simulink model "g1_walking"  (R2025b)
settings: Solver=daessc  StartTime=0.0  StopTime=4.8  MaxStep=0.0005  RelTol=1e-6  AbsTol=1e-8
model workspace (MAT data in the model file):
  g1_base_p0 = [0; 0; 0.8]
  g1_base_rpy0 = [0; 0; 0]
  g1_command_height = 0.8
  g1_forward_command = 0.1
  g1_gravity = [0 0 -9.81]
  g1_q0 = [-0.05; 0; 0; -0.05; 0; 0; 0.1; 0; 0; 0; 0; 0; 0; -0.05; 0; 0; -0.05; 0; 0; 0.1; 0; 0; 0; 0; 0; 0; 0; 0; 0]
  g1_qd0 = [0; 0; 0; 0; 0; 0; 0; 0; 0; 0; 0; 0; 0; 0; 0; 0; 0; 0; 0; 0; 0; 0; 0; 0; 0; 0; 0; 0; 0]
  g1_standing = 0
values from neighbouring files (symbols this model uses):
  g1_action_Ts = 0.002    [g1_data.sldd]
  g1_contact_threshold = 1.0    [g1_data.sldd]
  g1_cop_threshold = 5.0    [g1_data.sldd]
  g1_drive_Ts = 0.0005    [g1_data.sldd]
  g1_ground_height = 0.0    [g1_data.sldd]
  g1_limits = -0.87267 -0.2618 -1.0472 -2.5307 -0.5236 -2.7576 -0.087267 -3.0892 -1.5882 -2.618 -1.614429558 -1.972222054 -1.614429558 -0.87267 -0.2618 -1.0472 -2.5307 -2.9671 -2.7576 -0.087267 -3.0892 -2.2515 -2.618 -1.614429558 -1.972222054 -1.614429558 -0.52 -0.52 -2.618 0.5236 0.2618 2.0944 2.8798 2.9671 2.7576 2.8798 2.6704 2.2515 2.618 1.614429558 1.972222054 1.614429558 0.5236 0.2618 2.0944 2.8798 0.5236    [g1_data.sldd]
  g1_tau_max = 50.0 50.0 25.0 88.0 88.0 88.0 139.0 25.0 25.0 25.0 5.0 25.0 5.0 50.0 50.0 25.0 88.0 88.0 88.0 139.0 25.0 25.0 25.0 5.0 25.0 5.0 50.0 50.0 88.0    [g1_data.sldd]
undefined symbols (not defined in the file or in its folder): X, Y, Z
libraries: sm_lib x336, nesl_utility x122, simulink x1
(part 1 of 7)
Description:
  | Shared plant and drive model. Replace Planner and ReferenceGait model references through g1.walkingSimulation. Planner output 4 is RobotJointAction; output 3 is formulation-specific diagnostics.
settings Model: DataDictionary=g1_data.sldd  EnableAccessToBaseWorkspace=off  Creator=enoch  LastModifiedBy=enoch
settings DataIOCC: OutputOption=SpecifiedOutputTimes  OutputTimes=0:g1_drive_Ts:0.02

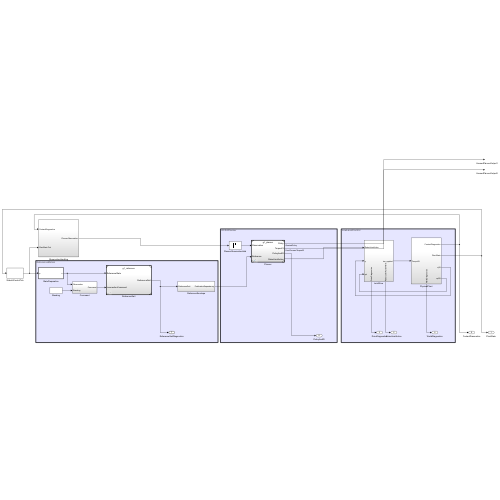
[thumbnail: Simulink's stored preview of the top-level diagram]
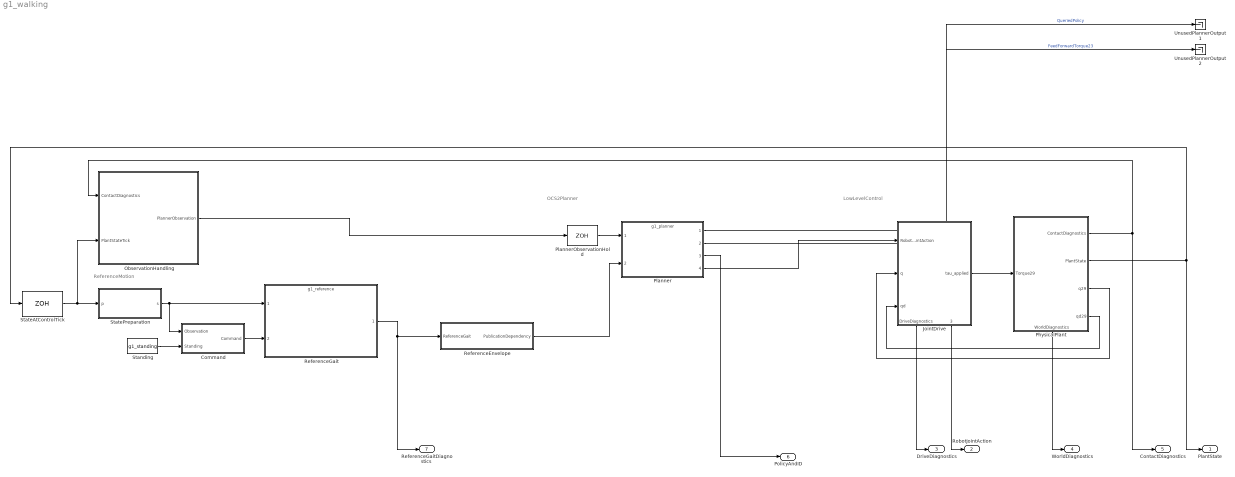
== system g1_walking ==
  note: ReferenceMotion
  note: LowLevelControl
  note: OCS2Planner
  Command : Subsystem
  JointDrive : Subsystem
      settings: PortSchema="{\"entries\":[{\"content\":{\"sides\":[{\"content\":{\"connectorIds\":[\"In1\",\"In2\",\"In3\"]},\"type\":\"ConnectorPlacement.EquallySpacedRectSide\",\"uuid\":\"f196539c-7e0c-46e2-93d7-b8c004bee5d8\"},{\"content\":{\"connectorIds\":[\"Out1\"],\"side\":\"RIGHT\"},\"type\":\"ConnectorPlacement.EquallySpacedRectSide\",\"uuid\":\"4b73e834-ba5b-4df9-9b66-b747ae678424\"},{\"content\":{\"side\":\"TOP\"},\"type\":\"ConnectorPlacement.EquallySpacedRectSide\",\"uuid\":\"8c147668-cc90-4ba0-ab32-ff0289ec25b5\"},{\"content\":{\"connectorIds\":[\"Out2\",\"Out3\"],\"side\":\"BOTTOM\"},\"type\":\"ConnectorPlacement.EquallySpacedRectSide\",\"uuid\":\"b0799187-69af-40f2-9cd9-a207ec5d2f97\"}]},\"type\":\"ConnectorPlacement.EquallySpacedConnector\",\"uuid\":\"1593d681-e81c-4265-8f53-8017c9fb3c0e\"}],\"packageUris\":[\"http://schema.mathworks.com/mf0/Connector/R2020b\"],\"version\":\"1.0\"}"
  ObservationHandling : Subsystem
  PhysicalPlant : Subsystem
      settings: PortSchema="{\"entries\":[{\"content\":{\"sides\":[{\"content\":{\"connectorIds\":[\"In1\"]},\"type\":\"ConnectorPlacement.EquallySpacedRectSide\",\"uuid\":\"a507f4f5-ee15-4ea4-b4de-ee914fc00dbd\"},{\"content\":{\"connectorIds\":[\"Out1\",\"Out2\",\"Out3\",\"Out4\"],\"side\":\"RIGHT\"},\"type\":\"ConnectorPlacement.EquallySpacedRectSide\",\"uuid\":\"97922e05-916d-4b63-ade6-e6a31880c11e\"},{\"content\":{\"side\":\"TOP\"},\"type\":\"ConnectorPlacement.EquallySpacedRectSide\",\"uuid\":\"4b0f9a05-b660-4a8d-9924-e10bf0b50292\"},{\"content\":{\"connectorIds\":[\"Out5\"],\"side\":\"BOTTOM\"},\"type\":\"ConnectorPlacement.EquallySpacedRectSide\",\"uuid\":\"154f9ed9-5c0e-4660-9782-88fd8999bb78\"}]},\"type\":\"ConnectorPlacement.EquallySpacedConnector\",\"uuid\":\"39aad6ea-4337-4531-a906-2cb26f9d93f7\"}],\"packageUris\":[\"http://schema.mathworks.com/mf0/Connector/R2020b\"],\"version\":\"1.0\"}"
  Planner : ModelReference  ModelNameDialog=g1_planner  SimulationMode=Normal  ModelReferenceVersion=1.16
  PlannerObservationHold : ZeroOrderHold  SampleTime=.002
  ReferenceEnvelope : Subsystem  Description=Flatten the coherent reference bus for the direct in-process planner call. No transport or file publication.
  ReferenceGait : ModelReference  Description=Authoritative command processing, target generation and gait state machine.  ModelNameDialog=g1_reference  SimulationMode=Normal  ModelReferenceVersion=1.19
  Standing : Constant  Value=g1_standing
  StateAtControlTick : ZeroOrderHold  SampleTime=.002
  StatePreparation : MATLAB Function  TreatAsAtomicUnit=on
  UnusedPlannerOutput1 : Terminator
  UnusedPlannerOutput2 : Terminator
  PlantState : Outport
  RobotJointAction : Outport  Port=2
  DriveDiagnostics : Outport  Port=3
  WorldDiagnostics : Outport  Port=4
  ContactDiagnostics : Outport  Port=5
  PolicyAndID : Outport  Port=6
  ReferenceGaitDiagnostics : Outport  Port=7  OutDataTypeStr=Bus: ReferenceGait  BusOutputAsStruct=on
  wires:
  PhysicalPlant/2(PlantState) -> StateAtControlTick/1, PlantState/1
  StateAtControlTick/1 -> ObservationHandling/2(PlantStateTick), StatePreparation/1(p)
  StatePreparation/1(s) -> ReferenceGait/1, Command/1(Observation)
  Standing/1 -> Command/2(Standing)
  Command/1(Command) -> ReferenceGait/2
  PhysicalPlant/1(ContactDiagnostics) -> ContactDiagnostics/1, ObservationHandling/1(ContactDiagnostics)
  PhysicalPlant/3(q29) -> JointDrive/2(q)
  PhysicalPlant/4(qd29) -> JointDrive/3(qd)
  JointDrive/1(tau_applied) -> PhysicalPlant/1(Torque29)
  JointDrive/3(RobotJointActionHeld) -> RobotJointAction/1
  JointDrive/2(DriveDiagnostics) -> DriveDiagnostics/1
  PhysicalPlant/5(WorldDiagnostics) -> WorldDiagnostics/1
  Planner/3 -> PolicyAndID/1
  ReferenceEnvelope/1(PublicationDependency) -> Planner/2
  PlannerObservationHold/1 -> Planner/1
  ObservationHandling/1(PlannerObservation) -> PlannerObservationHold/1
  ReferenceGait/1 -> ReferenceEnvelope/1(ReferenceGait), ReferenceGaitDiagnostics/1
  Planner/4 -> JointDrive/1(RobotJointAction)
  Planner/1 -> UnusedPlannerOutput1/1  "QueriedPolicy"
  Planner/2 -> UnusedPlannerOutput2/1  "FeedForwardTorque23"

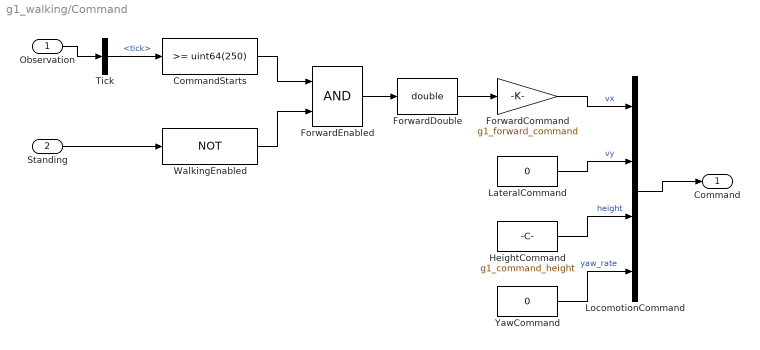
== system g1_walking/Command ==
  Observation : Inport  OutDataTypeStr=Bus: ReferenceObservation
  Standing : Inport  Port=2
  CommandStarts : simulink/Logic and Bit Operations/Compare To Constant  relop=>=  const=uint64(250)  OutDataTypeStr=boolean
  ForwardCommand : Gain  Gain=g1_forward_command
  ForwardDouble : DataTypeConversion  OutDataTypeStr=double  SaturateOnIntegerOverflow=off  RndMeth=Floor
  ForwardEnabled : Logic  AllPortsSameDT=off  OutDataTypeStr=boolean
  HeightCommand : Constant  Value=g1_command_height
  LateralCommand : Constant  Value=0
  LocomotionCommand : BusCreator  Inputs=4  OutDataTypeStr=Bus: LocomotionCommand  NonVirtualBus=on
  Tick : BusSelector  OutputSignals=tick
  WalkingEnabled : Logic  Operator=NOT  Inputs=1  AllPortsSameDT=off  OutDataTypeStr=boolean
  YawCommand : Constant  Value=0
  Command : Outport
  wires:
  Observation/1 -> Tick/1
  Tick/1 -> CommandStarts/1  "<tick>"
  Standing/1 -> WalkingEnabled/1
  CommandStarts/1 -> ForwardEnabled/1
  WalkingEnabled/1 -> ForwardEnabled/2
  ForwardEnabled/1 -> ForwardDouble/1
  ForwardDouble/1 -> ForwardCommand/1
  LocomotionCommand/1 -> Command/1
  ForwardCommand/1 -> LocomotionCommand/1  "vx"
  LateralCommand/1 -> LocomotionCommand/2  "vy"
  HeightCommand/1 -> LocomotionCommand/3  "height"
  YawCommand/1 -> LocomotionCommand/4  "yaw_rate"

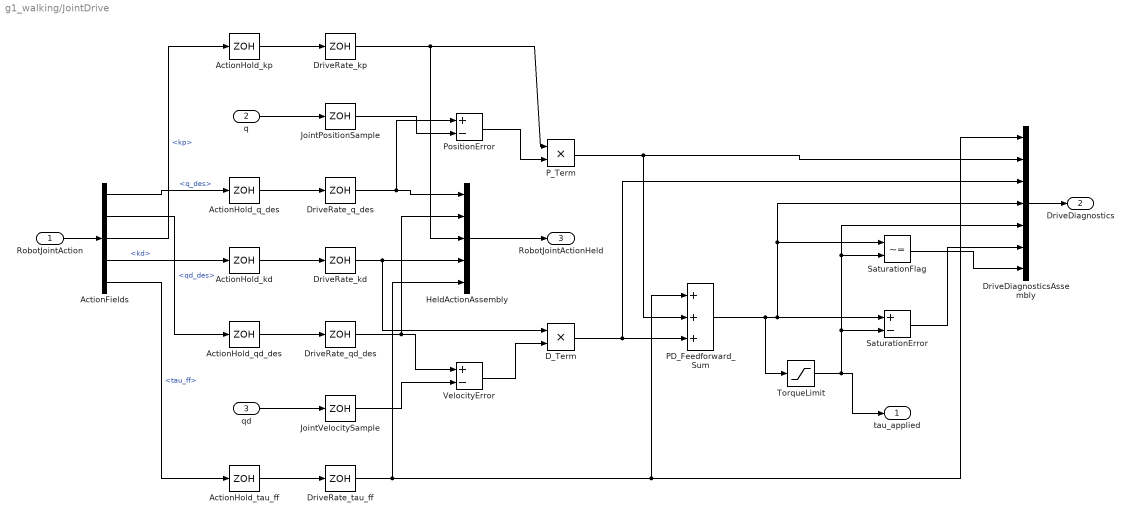
== system g1_walking/JointDrive ==
  RobotJointAction : Inport  OutDataTypeStr=Bus: RobotJointAction
  q : Inport  Port=2  PortDimensions=29
  qd : Inport  Port=3  PortDimensions=29
  ActionFields : BusSelector  OutputSignals=q_des,qd_des,kp,kd,tau_ff
  ActionHold_kd : ZeroOrderHold  SampleTime=g1_action_Ts
  ActionHold_kp : ZeroOrderHold  SampleTime=g1_action_Ts
  ActionHold_q_des : ZeroOrderHold  SampleTime=g1_action_Ts
  ActionHold_qd_des : ZeroOrderHold  SampleTime=g1_action_Ts
  ActionHold_tau_ff : ZeroOrderHold  SampleTime=g1_action_Ts
  D_Term : Product  Inputs=**
  DriveDiagnosticsAssembly : BusCreator  Inputs=7  OutDataTypeStr=Bus: DriveDiagnostics  NonVirtualBus=on
      settings: InheritFromInputs=off
  DriveRate_kd : ZeroOrderHold  SampleTime=g1_drive_Ts
  DriveRate_kp : ZeroOrderHold  SampleTime=g1_drive_Ts
  DriveRate_q_des : ZeroOrderHold  SampleTime=g1_drive_Ts
  DriveRate_qd_des : ZeroOrderHold  SampleTime=g1_drive_Ts
  DriveRate_tau_ff : ZeroOrderHold  SampleTime=g1_drive_Ts
  HeldActionAssembly : BusCreator  Inputs=5  OutDataTypeStr=Bus: RobotJointAction  NonVirtualBus=on
      settings: InheritFromInputs=off
  JointPositionSample : ZeroOrderHold  SampleTime=g1_drive_Ts
  JointVelocitySample : ZeroOrderHold  SampleTime=g1_drive_Ts
  PD_Feedforward_Sum : Sum  Inputs=+++
  P_Term : Product  Inputs=**
  PositionError : Sum  Inputs=+-
  SaturationError : Sum  Inputs=+-
  SaturationFlag : RelationalOperator  Operator=~=  OutDataTypeStr=boolean  RndMeth=Simplest  InputSameDT=off
  TorqueLimit : Saturate  UpperLimit=g1_tau_max  LowerLimit=-g1_tau_max
  VelocityError : Sum  Inputs=+-
  tau_applied : Outport
  DriveDiagnostics : Outport  Port=2
  RobotJointActionHeld : Outport  Port=3
  wires:
  DriveDiagnosticsAssembly/1 -> DriveDiagnostics/1
  HeldActionAssembly/1 -> RobotJointActionHeld/1
  SaturationFlag/1 -> DriveDiagnosticsAssembly/7
  SaturationError/1 -> DriveDiagnosticsAssembly/6
  TorqueLimit/1 -> SaturationFlag/2, DriveDiagnosticsAssembly/5, SaturationError/2, tau_applied/1
  PD_Feedforward_Sum/1 -> SaturationFlag/1, DriveDiagnosticsAssembly/4, SaturationError/1, TorqueLimit/1
  D_Term/1 -> PD_Feedforward_Sum/3, DriveDiagnosticsAssembly/3
  P_Term/1 -> PD_Feedforward_Sum/2, DriveDiagnosticsAssembly/2
  VelocityError/1 -> D_Term/2
  PositionError/1 -> P_Term/2
  JointVelocitySample/1 -> VelocityError/2
  JointPositionSample/1 -> PositionError/2
  DriveRate_tau_ff/1 -> PD_Feedforward_Sum/1, DriveDiagnosticsAssembly/1, HeldActionAssembly/5
  ActionHold_tau_ff/1 -> DriveRate_tau_ff/1
  ActionFields/5 -> ActionHold_tau_ff/1  "<tau_ff>"
  DriveRate_kd/1 -> HeldActionAssembly/4, D_Term/1
  ActionHold_kd/1 -> DriveRate_kd/1
  ActionFields/4 -> ActionHold_kd/1  "<kd>"
  DriveRate_kp/1 -> HeldActionAssembly/3, P_Term/1
  ActionHold_kp/1 -> DriveRate_kp/1
  ActionFields/3 -> ActionHold_kp/1  "<kp>"
  DriveRate_qd_des/1 -> HeldActionAssembly/2, VelocityError/1
  ActionHold_qd_des/1 -> DriveRate_qd_des/1
  ActionFields/2 -> ActionHold_qd_des/1  "<qd_des>"
  DriveRate_q_des/1 -> HeldActionAssembly/1, PositionError/1
  ActionHold_q_des/1 -> DriveRate_q_des/1
  ActionFields/1 -> ActionHold_q_des/1  "<q_des>"
  qd/1 -> JointVelocitySample/1
  q/1 -> JointPositionSample/1
  RobotJointAction/1 -> ActionFields/1

== system g1_walking/ObservationHandling ==
  ContactDiagnostics : Inport
  PlantStateTick : Inport  Port=2
  ContactDouble1 : DataTypeConversion  OutDataTypeStr=double  SaturateOnIntegerOverflow=off  RndMeth=Floor
  ContactDouble2 : DataTypeConversion  OutDataTypeStr=double  SaturateOnIntegerOverflow=off  RndMeth=Floor
  MeasuredContact : BusSelector  OutputSignals=Left.in_contact,Right.in_contact
  ObservationFields : BusSelector  OutputSignals=sim_time,base_position_world,base_orientation_wxyz,base_linear_velocity_local,base_angular_velocity_local,q,qd
  ObservationVector : Mux  Inputs=9
  PlannerObservation : Outport
  wires:
  ObservationFields/6 -> ObservationVector/6  "<q>"
  ContactDouble1/1 -> ObservationVector/8
  ObservationFields/1 -> ObservationVector/1  "<sim_time>"
  PlantStateTick/1 -> ObservationFields/1
  ObservationFields/2 -> ObservationVector/2  "<base_position_world>"
  MeasuredContact/1 -> ContactDouble1/1  "<in_contact>"
  ObservationFields/3 -> ObservationVector/3  "<base_orientation_wxyz>"
  ContactDiagnostics/1 -> MeasuredContact/1
  ContactDouble2/1 -> ObservationVector/9
  MeasuredContact/2 -> ContactDouble2/1  "<in_contact>"
  ObservationFields/4 -> ObservationVector/4  "<base_linear_velocity_local>"
  ObservationFields/5 -> ObservationVector/5  "<base_angular_velocity_local>"
  ObservationFields/7 -> ObservationVector/7  "<qd>"
  ObservationVector/1 -> PlannerObservation/1

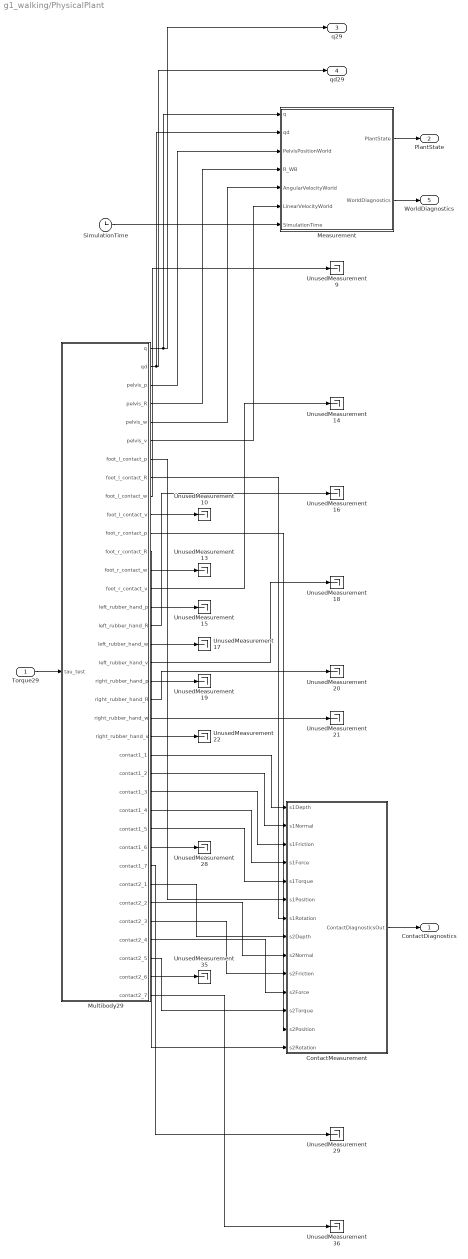
== system g1_walking/PhysicalPlant ==
  Torque29 : Inport
  ContactMeasurement : Subsystem
  Measurement : Subsystem
  Multibody29 : Subsystem
  SimulationTime : Clock
  UnusedMeasurement{9..10,13..22,28..29,35..36} (16 alike) : Terminator
  ContactDiagnostics : Outport
  PlantState : Outport  Port=2
  q29 : Outport  Port=3
  qd29 : Outport  Port=4
  WorldDiagnostics : Outport  Port=5
  wires:
  Torque29/1 -> Multibody29/1(tau_test)
  Multibody29/1(q) -> q29/1, Measurement/1(q)
  Multibody29/2(qd) -> qd29/1, Measurement/2(qd)
  Multibody29/3(pelvis_p) -> Measurement/3(PelvisPositionWorld)
  Multibody29/4(pelvis_R) -> Measurement/4(R_WB)
  Multibody29/5(pelvis_w) -> Measurement/5(AngularVelocityWorld)
  Multibody29/6(pelvis_v) -> Measurement/6(LinearVelocityWorld)
  SimulationTime/1 -> Measurement/7(SimulationTime)
  Multibody29/23(contact1_1) -> ContactMeasurement/1(s1Depth)
  Multibody29/24(contact1_2) -> ContactMeasurement/2(s1Normal)
  Multibody29/25(contact1_3) -> ContactMeasurement/3(s1Friction)
  Multibody29/26(contact1_4) -> ContactMeasurement/4(s1Force)
  Multibody29/27(contact1_5) -> ContactMeasurement/5(s1Torque)
  Multibody29/7(foot_l_contact_p) -> ContactMeasurement/6(s1Position)
  Multibody29/8(foot_l_contact_R) -> ContactMeasurement/7(s1Rotation)
  Multibody29/30(contact2_1) -> ContactMeasurement/8(s2Depth)
  Multibody29/31(contact2_2) -> ContactMeasurement/9(s2Normal)
  Multibody29/32(contact2_3) -> ContactMeasurement/10(s2Friction)
  Multibody29/33(contact2_4) -> ContactMeasurement/11(s2Force)
  Multibody29/34(contact2_5) -> ContactMeasurement/12(s2Torque)
  Multibody29/11(foot_r_contact_p) -> ContactMeasurement/13(s2Position)
  Multibody29/12(foot_r_contact_R) -> ContactMeasurement/14(s2Rotation)
  Multibody29/9(foot_l_contact_w) -> UnusedMeasurement9/1
  Multibody29/10(foot_l_contact_v) -> UnusedMeasurement10/1
  Multibody29/13(foot_r_contact_w) -> UnusedMeasurement13/1
  Multibody29/14(foot_r_contact_v) -> UnusedMeasurement14/1
  Multibody29/15(left_rubber_hand_p) -> UnusedMeasurement15/1
  Multibody29/16(left_rubber_hand_R) -> UnusedMeasurement16/1
  Multibody29/17(left_rubber_hand_w) -> UnusedMeasurement17/1
  Multibody29/18(left_rubber_hand_v) -> UnusedMeasurement18/1
  Multibody29/19(right_rubber_hand_p) -> UnusedMeasurement19/1
  Multibody29/20(right_rubber_hand_R) -> UnusedMeasurement20/1
  Multibody29/21(right_rubber_hand_w) -> UnusedMeasurement21/1
  Multibody29/22(right_rubber_hand_v) -> UnusedMeasurement22/1
  Multibody29/28(contact1_6) -> UnusedMeasurement28/1
  Multibody29/29(contact1_7) -> UnusedMeasurement29/1
  Multibody29/35(contact2_6) -> UnusedMeasurement35/1
  Multibody29/36(contact2_7) -> UnusedMeasurement36/1
  Measurement/1(PlantState) -> PlantState/1
  Measurement/2(WorldDiagnostics) -> WorldDiagnostics/1
  ContactMeasurement/1(ContactDiagnosticsOut) -> ContactDiagnostics/1

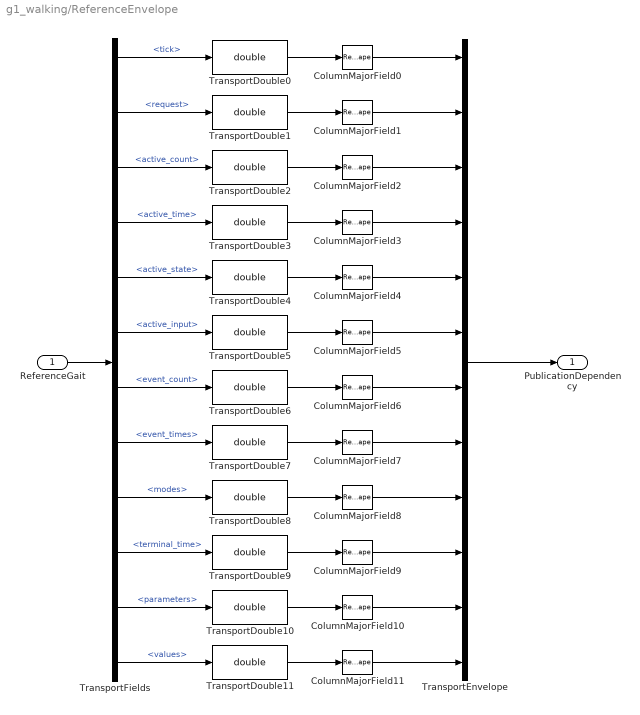
== system g1_walking/ReferenceEnvelope ==
  ReferenceGait : Inport  OutDataTypeStr=Bus: ReferenceGait
  ColumnMajorField{0..11} (12 alike) : Reshape
  TransportDouble{0..11} (12 alike) : DataTypeConversion  OutDataTypeStr=double  SaturateOnIntegerOverflow=off  RndMeth=Floor
  TransportEnvelope : Mux  Inputs=12
  TransportFields : BusSelector  OutputSignals=command.tick,command.request,target.active_count,target.active_time,target.active_state,target.active_input,schedule.event_count,schedule.event_times,schedule.modes,schedule.terminal_time,swing.parameters,command.values
  PublicationDependency : Outport  OutDataTypeStr=double
  wires:
  ColumnMajorField11/1 -> TransportEnvelope/12
  TransportDouble11/1 -> ColumnMajorField11/1
  TransportFields/12 -> TransportDouble11/1  "<values>"
  ColumnMajorField10/1 -> TransportEnvelope/11
  TransportDouble10/1 -> ColumnMajorField10/1
  TransportFields/11 -> TransportDouble10/1  "<parameters>"
  ColumnMajorField9/1 -> TransportEnvelope/10
  TransportDouble9/1 -> ColumnMajorField9/1
  TransportFields/10 -> TransportDouble9/1  "<terminal_time>"
  ColumnMajorField8/1 -> TransportEnvelope/9
  TransportDouble8/1 -> ColumnMajorField8/1
  TransportFields/9 -> TransportDouble8/1  "<modes>"
  ColumnMajorField7/1 -> TransportEnvelope/8
  TransportDouble7/1 -> ColumnMajorField7/1
  TransportFields/8 -> TransportDouble7/1  "<event_times>"
  ColumnMajorField6/1 -> TransportEnvelope/7
  TransportDouble6/1 -> ColumnMajorField6/1
  TransportFields/7 -> TransportDouble6/1  "<event_count>"
  ColumnMajorField5/1 -> TransportEnvelope/6
  TransportDouble5/1 -> ColumnMajorField5/1
  TransportFields/6 -> TransportDouble5/1  "<active_input>"
  ColumnMajorField4/1 -> TransportEnvelope/5
  TransportDouble4/1 -> ColumnMajorField4/1
  TransportFields/5 -> TransportDouble4/1  "<active_state>"
  ColumnMajorField3/1 -> TransportEnvelope/4
  TransportDouble3/1 -> ColumnMajorField3/1
  TransportFields/4 -> TransportDouble3/1  "<active_time>"
  ColumnMajorField2/1 -> TransportEnvelope/3
  TransportDouble2/1 -> ColumnMajorField2/1
  TransportFields/3 -> TransportDouble2/1  "<active_count>"
  ColumnMajorField1/1 -> TransportEnvelope/2
  TransportDouble1/1 -> ColumnMajorField1/1
  TransportFields/2 -> TransportDouble1/1  "<request>"
  ColumnMajorField0/1 -> TransportEnvelope/1
  TransportDouble0/1 -> ColumnMajorField0/1
  TransportFields/1 -> TransportDouble0/1  "<tick>"
  ReferenceGait/1 -> TransportFields/1
  TransportEnvelope/1 -> PublicationDependency/1

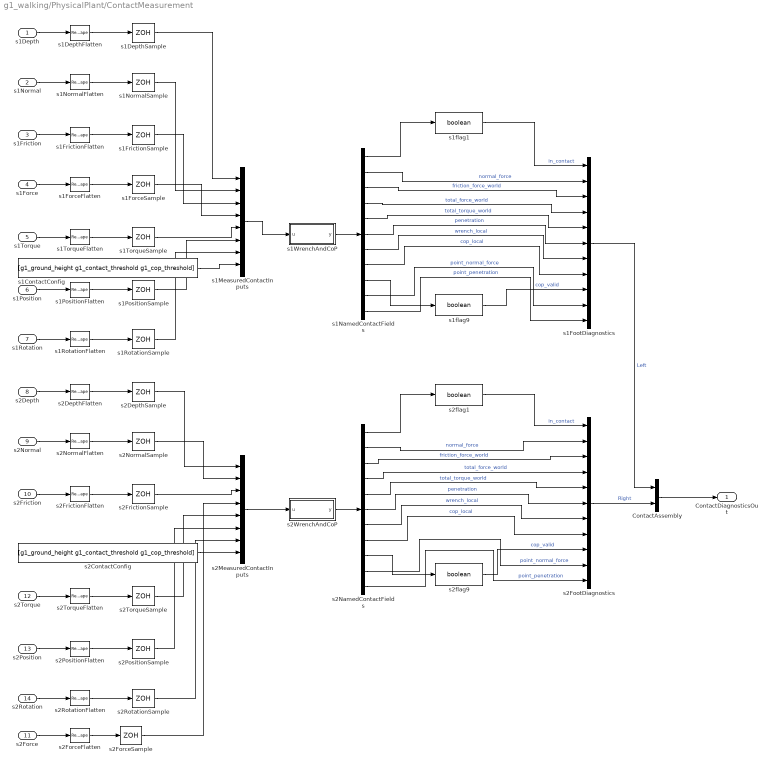
== system g1_walking/PhysicalPlant/ContactMeasurement ==
  s1Depth : Inport
  s1Normal : Inport  Port=2
  s1Friction : Inport  Port=3
  s1Force : Inport  Port=4
  s1Torque : Inport  Port=5
  s1Position : Inport  Port=6
  s1Rotation : Inport  Port=7
  s2Depth : Inport  Port=8
  s2Normal : Inport  Port=9
  s2Friction : Inport  Port=10
  s2Force : Inport  Port=11
  s2Torque : Inport  Port=12
  s2Position : Inport  Port=13
  s2Rotation : Inport  Port=14
  ContactAssembly : BusCreator  Inputs=2  OutDataTypeStr=Bus: ContactDiagnostics  NonVirtualBus=on
  s1ContactConfig : Constant  Value=[g1_ground_height g1_contact_threshold g1_cop_threshold]
  s1DepthFlatten : Reshape
  s1DepthSample : ZeroOrderHold  SampleTime=g1_drive_Ts
  s1FootDiagnostics : BusCreator  Inputs=11  OutDataTypeStr=Bus: FootContactDiagnostics  NonVirtualBus=on
  s1ForceFlatten : Reshape
  s1ForceSample : ZeroOrderHold  SampleTime=g1_drive_Ts
  s1FrictionFlatten : Reshape
  s1FrictionSample : ZeroOrderHold  SampleTime=g1_drive_Ts
  s1MeasuredContactInputs : Mux  Inputs=8
  s1NamedContactFields : Demux  Outputs=[1 1 3 3 3 1 6 2 1 4 4]
  s1NormalFlatten : Reshape
  s1NormalSample : ZeroOrderHold  SampleTime=g1_drive_Ts
  s1PositionFlatten : Reshape
  s1PositionSample : ZeroOrderHold  SampleTime=g1_drive_Ts
  s1RotationFlatten : Reshape
  s1RotationSample : ZeroOrderHold  SampleTime=g1_drive_Ts
  s1TorqueFlatten : Reshape
  s1TorqueSample : ZeroOrderHold  SampleTime=g1_drive_Ts
  s1WrenchAndCoP : MATLAB Function  TreatAsAtomicUnit=on
  s1flag1 : DataTypeConversion  OutDataTypeStr=boolean  SaturateOnIntegerOverflow=off  RndMeth=Floor
  s1flag9 : DataTypeConversion  OutDataTypeStr=boolean  SaturateOnIntegerOverflow=off  RndMeth=Floor
  s2ContactConfig : Constant  Value=[g1_ground_height g1_contact_threshold g1_cop_threshold]
  s2DepthFlatten : Reshape
  s2DepthSample : ZeroOrderHold  SampleTime=g1_drive_Ts
  s2FootDiagnostics : BusCreator  Inputs=11  OutDataTypeStr=Bus: FootContactDiagnostics  NonVirtualBus=on
  s2ForceFlatten : Reshape
  s2ForceSample : ZeroOrderHold  SampleTime=g1_drive_Ts
  s2FrictionFlatten : Reshape
  s2FrictionSample : ZeroOrderHold  SampleTime=g1_drive_Ts
  s2MeasuredContactInputs : Mux  Inputs=8
  s2NamedContactFields : Demux  Outputs=[1 1 3 3 3 1 6 2 1 4 4]
  s2NormalFlatten : Reshape
  s2NormalSample : ZeroOrderHold  SampleTime=g1_drive_Ts
  s2PositionFlatten : Reshape
  s2PositionSample : ZeroOrderHold  SampleTime=g1_drive_Ts
  s2RotationFlatten : Reshape
  s2RotationSample : ZeroOrderHold  SampleTime=g1_drive_Ts
  s2TorqueFlatten : Reshape
  s2TorqueSample : ZeroOrderHold  SampleTime=g1_drive_Ts
  s2WrenchAndCoP : MATLAB Function  TreatAsAtomicUnit=on
  s2flag1 : DataTypeConversion  OutDataTypeStr=boolean  SaturateOnIntegerOverflow=off  RndMeth=Floor
  s2flag9 : DataTypeConversion  OutDataTypeStr=boolean  SaturateOnIntegerOverflow=off  RndMeth=Floor
  ContactDiagnosticsOut : Outport  OutDataTypeStr=Bus: ContactDiagnostics
  wires:
  s2FootDiagnostics/1 -> ContactAssembly/2  "Right"
  s2NamedContactFields/11 -> s2FootDiagnostics/11  "point_penetration"
  s2NamedContactFields/10 -> s2FootDiagnostics/10  "point_normal_force"
  s2flag9/1 -> s2FootDiagnostics/9  "cop_valid"
  s2NamedContactFields/9 -> s2flag9/1
  s2NamedContactFields/8 -> s2FootDiagnostics/8  "cop_local"
  s2NamedContactFields/7 -> s2FootDiagnostics/7  "wrench_local"
  s2NamedContactFields/6 -> s2FootDiagnostics/6  "penetration"
  s2NamedContactFields/5 -> s2FootDiagnostics/5  "total_torque_world"
  s2NamedContactFields/4 -> s2FootDiagnostics/4  "total_force_world"
  s2NamedContactFields/3 -> s2FootDiagnostics/3  "friction_force_world"
  s2NamedContactFields/2 -> s2FootDiagnostics/2  "normal_force"
  s2flag1/1 -> s2FootDiagnostics/1  "in_contact"
  s2NamedContactFields/1 -> s2flag1/1
  s2RotationSample/1 -> s2MeasuredContactInputs/7
  s2RotationFlatten/1 -> s2RotationSample/1
  s2Rotation/1 -> s2RotationFlatten/1
  s2PositionSample/1 -> s2MeasuredContactInputs/6
  s2PositionFlatten/1 -> s2PositionSample/1
  s2Position/1 -> s2PositionFlatten/1
  s2TorqueSample/1 -> s2MeasuredContactInputs/5
  s2TorqueFlatten/1 -> s2TorqueSample/1
  s2Torque/1 -> s2TorqueFlatten/1
  s2FrictionSample/1 -> s2MeasuredContactInputs/3
  s2FrictionFlatten/1 -> s2FrictionSample/1
  s2Friction/1 -> s2FrictionFlatten/1
  s2NormalSample/1 -> s2MeasuredContactInputs/2
  s2NormalFlatten/1 -> s2NormalSample/1
  s2Normal/1 -> s2NormalFlatten/1
  s2DepthSample/1 -> s2MeasuredContactInputs/1
  s2DepthFlatten/1 -> s2DepthSample/1
  s2Depth/1 -> s2DepthFlatten/1
  s1FootDiagnostics/1 -> ContactAssembly/1  "Left"
  s1NamedContactFields/11 -> s1FootDiagnostics/11  "point_penetration"
  s1NamedContactFields/10 -> s1FootDiagnostics/10  "point_normal_force"
  s1flag9/1 -> s1FootDiagnostics/9  "cop_valid"
  s1NamedContactFields/9 -> s1flag9/1
  s1NamedContactFields/8 -> s1FootDiagnostics/8  "cop_local"
  s1NamedContactFields/7 -> s1FootDiagnostics/7  "wrench_local"
  s1NamedContactFields/6 -> s1FootDiagnostics/6  "penetration"
  s1NamedContactFields/5 -> s1FootDiagnostics/5  "total_torque_world"
  s1NamedContactFields/4 -> s1FootDiagnostics/4  "total_force_world"
  s1NamedContactFields/3 -> s1FootDiagnostics/3  "friction_force_world"
  s1NamedContactFields/2 -> s1FootDiagnostics/2  "normal_force"
  s1flag1/1 -> s1FootDiagnostics/1  "in_contact"
  s1NamedContactFields/1 -> s1flag1/1
  s1RotationSample/1 -> s1MeasuredContactInputs/7
  s1RotationFlatten/1 -> s1RotationSample/1
  s1Rotation/1 -> s1RotationFlatten/1
  s1PositionSample/1 -> s1MeasuredContactInputs/6
  s1PositionFlatten/1 -> s1PositionSample/1
  s1Position/1 -> s1PositionFlatten/1
  s1TorqueSample/1 -> s1MeasuredContactInputs/5
  s1TorqueFlatten/1 -> s1TorqueSample/1
  s1Torque/1 -> s1TorqueFlatten/1
  s1ForceSample/1 -> s1MeasuredContactInputs/4
  s1ForceFlatten/1 -> s1ForceSample/1
  s1Force/1 -> s1ForceFlatten/1
  s1FrictionSample/1 -> s1MeasuredContactInputs/3
  s1FrictionFlatten/1 -> s1FrictionSample/1
  s1Friction/1 -> s1FrictionFlatten/1
  s1NormalSample/1 -> s1MeasuredContactInputs/2
  s1NormalFlatten/1 -> s1NormalSample/1
  s1Normal/1 -> s1NormalFlatten/1
  s1DepthSample/1 -> s1MeasuredContactInputs/1
  s1DepthFlatten/1 -> s1DepthSample/1
  s1Depth/1 -> s1DepthFlatten/1
  ContactAssembly/1 -> ContactDiagnosticsOut/1
  s2ContactConfig/1 -> s2MeasuredContactInputs/8
  s1ContactConfig/1 -> s1MeasuredContactInputs/8
  s2Force/1 -> s2ForceFlatten/1
  s2ForceFlatten/1 -> s2ForceSample/1
  s2ForceSample/1 -> s2MeasuredContactInputs/4
  s1MeasuredContactInputs/1 -> s1WrenchAndCoP/1(u)
  s1WrenchAndCoP/1(y) -> s1NamedContactFields/1
  s2MeasuredContactInputs/1 -> s2WrenchAndCoP/1(u)
  s2WrenchAndCoP/1(y) -> s2NamedContactFields/1

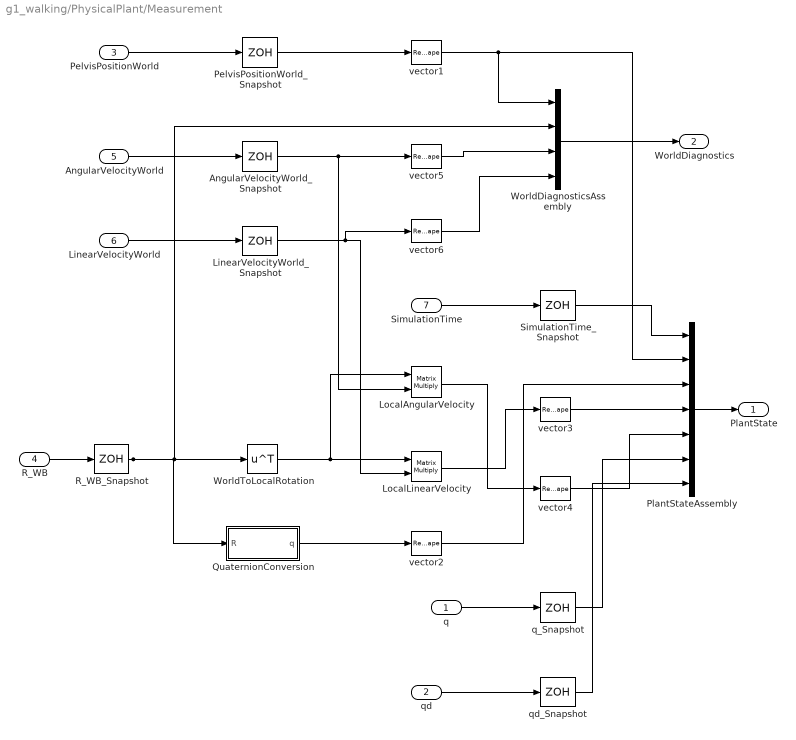
== system g1_walking/PhysicalPlant/Measurement ==
  q : Inport  PortDimensions=29
  qd : Inport  Port=2  PortDimensions=29
  PelvisPositionWorld : Inport  Port=3  PortDimensions=[3 1]
  R_WB : Inport  Port=4  PortDimensions=[3 3]
  AngularVelocityWorld : Inport  Port=5  PortDimensions=[3 1]
  LinearVelocityWorld : Inport  Port=6  PortDimensions=[3 1]
  SimulationTime : Inport  Port=7  PortDimensions=1
  AngularVelocityWorld_Snapshot : ZeroOrderHold  SampleTime=g1_drive_Ts
  LinearVelocityWorld_Snapshot : ZeroOrderHold  SampleTime=g1_drive_Ts
  LocalAngularVelocity : Product  Inputs=**  Multiplication=Matrix(*)
  LocalLinearVelocity : Product  Inputs=**  Multiplication=Matrix(*)
  PelvisPositionWorld_Snapshot : ZeroOrderHold  SampleTime=g1_drive_Ts
  PlantStateAssembly : BusCreator  Inputs=7  OutDataTypeStr=Bus: PlantState  NonVirtualBus=on
      settings: InheritFromInputs=off
  QuaternionConversion : MATLAB Function  TreatAsAtomicUnit=on
  R_WB_Snapshot : ZeroOrderHold  SampleTime=g1_drive_Ts
  SimulationTime_Snapshot : ZeroOrderHold  SampleTime=g1_drive_Ts
  WorldDiagnosticsAssembly : BusCreator  Inputs=4  OutDataTypeStr=Bus: WorldDiagnostics  NonVirtualBus=on
      settings: InheritFromInputs=off
  WorldToLocalRotation : Math  Operator=transpose
  q_Snapshot : ZeroOrderHold  SampleTime=g1_drive_Ts
  qd_Snapshot : ZeroOrderHold  SampleTime=g1_drive_Ts
  vector{1..6} (6 alike) : Reshape
  PlantState : Outport  OutDataTypeStr=Bus: PlantState
  WorldDiagnostics : Outport  Port=2  OutDataTypeStr=Bus: WorldDiagnostics
  wires:
  WorldDiagnosticsAssembly/1 -> WorldDiagnostics/1
  PlantStateAssembly/1 -> PlantState/1
  vector6/1 -> WorldDiagnosticsAssembly/4
  vector5/1 -> WorldDiagnosticsAssembly/3
  qd_Snapshot/1 -> PlantStateAssembly/7
  q_Snapshot/1 -> PlantStateAssembly/6
  vector4/1 -> PlantStateAssembly/5
  vector3/1 -> PlantStateAssembly/4
  vector2/1 -> PlantStateAssembly/3
  vector1/1 -> PlantStateAssembly/2, WorldDiagnosticsAssembly/1
  SimulationTime_Snapshot/1 -> PlantStateAssembly/1
  LocalAngularVelocity/1 -> vector4/1
  LocalLinearVelocity/1 -> vector3/1
  PelvisPositionWorld_Snapshot/1 -> vector1/1
  AngularVelocityWorld_Snapshot/1 -> vector5/1, LocalAngularVelocity/2
  LinearVelocityWorld_Snapshot/1 -> LocalLinearVelocity/2, vector6/1
  WorldToLocalRotation/1 -> LocalLinearVelocity/1, LocalAngularVelocity/1
  R_WB_Snapshot/1 -> WorldDiagnosticsAssembly/2, WorldToLocalRotation/1, QuaternionConversion/1(R)
  SimulationTime/1 -> SimulationTime_Snapshot/1
  LinearVelocityWorld/1 -> LinearVelocityWorld_Snapshot/1
  AngularVelocityWorld/1 -> AngularVelocityWorld_Snapshot/1
  R_WB/1 -> R_WB_Snapshot/1
  PelvisPositionWorld/1 -> PelvisPositionWorld_Snapshot/1
  qd/1 -> qd_Snapshot/1
  q/1 -> q_Snapshot/1
  QuaternionConversion/1(q) -> vector2/1
